simulink model "model"  (R2025b)
settings: Solver=VariableStepAuto  StartTime=0.0  StopTime=5  MaxStep=1e-5  RelTol=1e-5
values from neighbouring files (symbols this model uses):
  A = [0 1; 5 -3]    [init.m]
  b = [2; 5]    [init.m]
  K = Y * P^-1    [init.m]    (also in plots_3.m = r^-1 * b' * P*0.85; plots_4.m = r^-1 * b' * P)
  Q = [2 0; 0 3]    [init.m]    (also in plots_4.m = experiments{j, 1})
  r = 2    [init.m]    (also in plots_4.m = experiments{j, 2})
  x0 = [1;0]    [init.m]
settings Model: Creator=eva  LastModifiedBy=eva

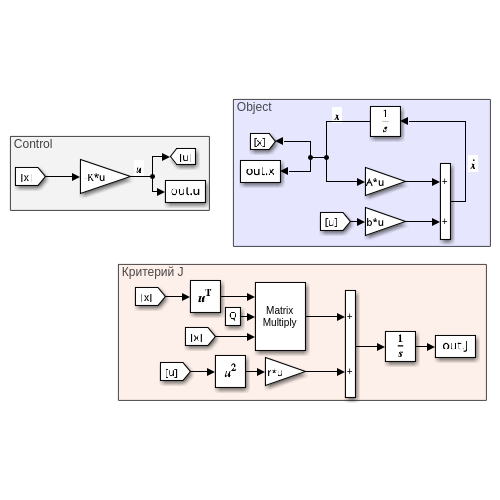
[thumbnail: Simulink's stored preview of the top-level diagram]
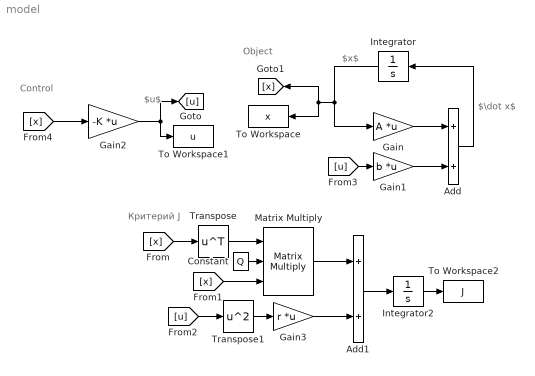
== system model ==
  note: Object
  note: Control
  note: Критерий J
  note: $x$
  note: $\dot x$
  note: $u$
  Add : Sum
  Add1 : Sum
  Constant : Constant  Value=Q
  Gain : Gain  Gain=A  Multiplication=Matrix(K*u)
  Gain1 : Gain  Gain=b  Multiplication=Matrix(K*u)
  Gain2 : Gain  Gain=-K  Multiplication=Matrix(K*u)
  Gain3 : Gain  Gain=r  Multiplication=Matrix(K*u)
  Integrator : Integrator  InitialCondition=x0
  Integrator2 : Integrator
  Matrix Multiply : Product  Inputs=3  Multiplication=Matrix(*)
  To Workspace : ToWorkspace  VariableName=x  SaveFormat=Structure With Time  SampleTime=-1
  To Workspace1 : ToWorkspace  VariableName=u  SaveFormat=Structure With Time  SampleTime=-1
  To Workspace2 : ToWorkspace  VariableName=J  SaveFormat=Structure With Time  SampleTime=-1
  Transpose : Math  Operator=transpose
  Transpose1 : Math  Operator=square
  wires:
  Gain/1 -> Add/1
  Gain1/1 -> Add/2
  Gain2/1 -> [u], To Workspace1/1
  Add/1 -> Integrator/1
  Integrator/1 -> Gain/1, [x], To Workspace/1
  [x] -> Transpose/1
  Transpose/1 -> Matrix Multiply/1
  Constant/1 -> Matrix Multiply/2
  Matrix Multiply/1 -> Add1/1
  [x] -> Matrix Multiply/3
  [u] -> Transpose1/1
  Transpose1/1 -> Gain3/1
  Gain3/1 -> Add1/2
  Add1/1 -> Integrator2/1
  Integrator2/1 -> To Workspace2/1
  [u] -> Gain1/1
  [x] -> Gain2/1
